simulink model "fw_vehicle_ctrl"  (R2026b)
settings: Solver=VariableStepAuto
undefined symbols (not defined in the file or in its folder): DiscIntNeverNeededParam, ImplementType, P, ShaddadMode, Ts
libraries: simulink x22, sl_discontinuities x6, slpidlib x1
settings Model: Creator=aomar  LastModifiedBy=aomar

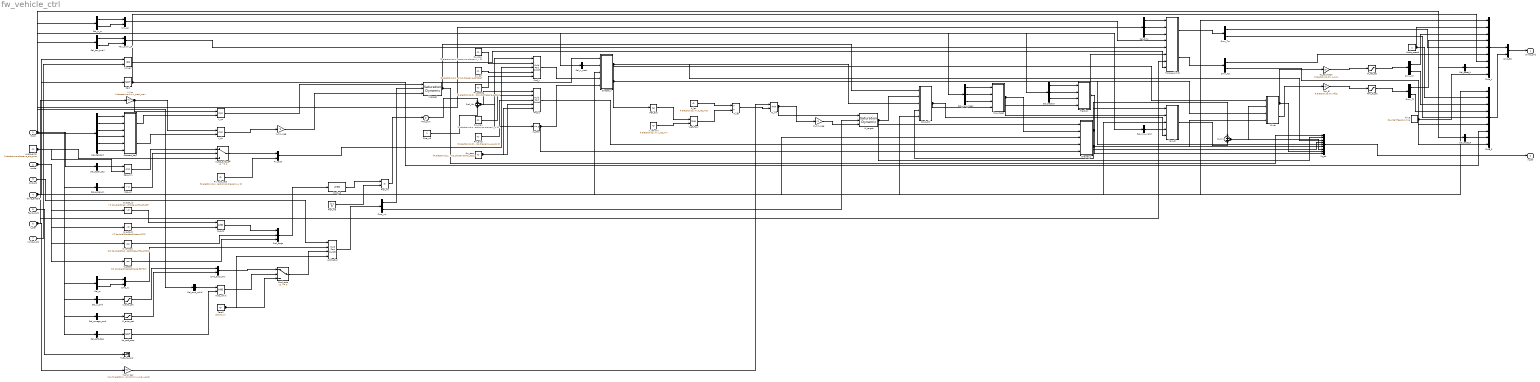
== system fw_vehicle_ctrl ==
  fw10 : Inport  SampleTime=Ts.ctrl
  mode : Inport  Port=2  OutDataTypeStr=uint8  SampleTime=Ts.ctrl
  cmd_src : Inport  Port=3  OutDataTypeStr=uint8  SampleTime=Ts.ctrl
  drive_enable : Inport  Port=4  OutDataTypeStr=boolean  SampleTime=Ts.ctrl
  fault_word : Inport  Port=5  OutDataTypeStr=uint32  SampleTime=Ts.ctrl
  k_der : Inport  Port=6  OutDataTypeStr=single  SampleTime=Ts.ctrl
  limits_hold : Inport  Port=7  OutDataTypeStr=boolean  SampleTime=Ts.ctrl
  A_acc_auto : Constant  Value=P.electronics.shaper.a_acc_auto  OutDataTypeStr=single  SampleTime=Ts.ctrl
  A_acc_auto_eff : Switch  Criteria=u2 ~= 0  SaturateOnIntegerOverflow=off  InputSameDT=off
  A_lat : Constant  Value=P.electronics.lim.a_lat_max  OutDataTypeStr=single  SampleTime=Ts.ctrl
  Alive : simulink/Sources/Counter Free-Running  NumBits=8  tsamp=Ts.ctrl
  Arbitration : MultiPortSwitch  DataPortOrder=Specify indices  DataPortIndices={1,2}  DataPortForDefault=Additional data port  DiagnosticForDefault=None  SaturateOnIntegerOverflow=off  InputSameDT=off
  Auto_valid : Logic  AllPortsSameDT=off  OutDataTypeStr=boolean
  Cap_min : MinMax  Inputs=2
  Cap_on : simulink/Logic and Bit Operations/Compare To Zero  relop=>  OutDataTypeStr=boolean
  Cmd_BC : BusCreator  Inputs=2  OutDataTypeStr=Bus: Bus_DriveCmd  NonVirtualBus=on
      settings: InheritFromInputs=off
  Cmd_auto : Switch  Criteria=u2 ~= 0  SaturateOnIntegerOverflow=off  InputSameDT=off
  Cmd_auto_raw : Concatenate
  Cmd_rc : Concatenate
  Cmd_still : Subsystem
  Cmd_vw : Demux  Outputs=2
  Descent_cap : Subsystem
  Dmx_Tf : Demux  Outputs=2
  Dmx_Tg : Demux  Outputs=2
  Dmx_Tm : Demux  Outputs=2
  Dmx_Wr : Demux  Outputs=2
  Is_auto : Logic  AllPortsSameDT=off  OutDataTypeStr=boolean
  Is_auto_hi : simulink/Logic and Bit Operations/Compare To Constant  relop=<=  const=double(ShaddadMode.AUTO)  OutDataTypeStr=boolean
  Is_auto_lo : simulink/Logic and Bit Operations/Compare To Constant  relop=>=  const=double(ShaddadMode.AUTO_START)  OutDataTypeStr=boolean
  Is_ctrlstop : simulink/Logic and Bit Operations/Compare To Constant  relop===  const=double(ShaddadMode.CTRL_STOP)  OutDataTypeStr=boolean
  Is_estop : simulink/Logic and Bit Operations/Compare To Constant  relop===  const=double(ShaddadMode.ESTOP)  OutDataTypeStr=boolean
  Is_stop : simulink/Logic and Bit Operations/Compare To Constant  relop=>=  const=3  OutDataTypeStr=boolean
  Lim_en : Logic  Operator=OR  AllPortsSameDT=off  OutDataTypeStr=boolean
  Mixer : Subsystem
  Mode_speed : Constant  OutDataTypeStr=uint8  SampleTime=Ts.ctrl
  No_soft_stop : Logic  Operator=NOT  Inputs=1  AllPortsSameDT=off  OutDataTypeStr=boolean
  One_u8 : Constant  OutDataTypeStr=uint8  SampleTime=Ts.ctrl
  Park : Logic  Operator=NOT  Inputs=1  AllPortsSameDT=off  OutDataTypeStr=boolean
  Prof_flags : Concatenate  NumInputs=3
  Prof_idx : Sum  OutDataTypeStr=uint8
  Prof_sum : Sum  Inputs=+  OutDataTypeStr=uint8
  Prof_u8 : DataTypeConversion  OutDataTypeStr=uint8  RndMeth=Round
  Prof_v : MultiPortSwitch  Inputs=4  DiagnosticForDefault=None  SaturateOnIntegerOverflow=off  InputSameDT=off
  Prof_w : MultiPortSwitch  Inputs=4  DiagnosticForDefault=None  SaturateOnIntegerOverflow=off  InputSameDT=off
  Prof_w8 : Constant  Value=[1 2 3]  OutDataTypeStr=uint8  SampleTime=Ts.ctrl
  Prof_wt : Product  Inputs=**  OutDataTypeStr=uint8
  Pv_auto : Concatenate
  Pv_auto_rest : Constant  Value=[P.electronics.shaper.a_dec_auto P.electronics.shaper.j_max P.electronics.shaper.K_v 0]  OutDataTypeStr=single  SampleTime=Ts.ctrl
  Pv_ctrl : Constant  Value=[P.electronics.shaper.a_ctrlstop P.electronics.shaper.a_ctrlstop P.electronics.shaper.j_stop P.electronics.shaper.K_v P.electronics.shaper.a_ctrlstop]  OutDataTypeStr=single  SampleTime=Ts.ctrl
  Pv_estop : Constant  Value=[P.electronics.shaper.a_estop P.electronics.shaper.a_estop P.electronics.shaper.j_stop P.electronics.shaper.K_v P.electronics.shaper.a_estop]  OutDataTypeStr=single  SampleTime=Ts.ctrl
  Pv_man : Constant  Value=[P.electronics.shaper.a_acc_man P.electronics.shaper.a_dec_man P.electronics.shaper.j_max P.electronics.shaper.K_v 0]  OutDataTypeStr=single  SampleTime=Ts.ctrl
  Pw_auto : Constant  Value=[P.electronics.shaper.alpha_auto P.electronics.shaper.alpha_auto P.electronics.shaper.jw_auto P.electronics.shaper.K_w_auto 0]  OutDataTypeStr=single  SampleTime=Ts.ctrl
  Pw_man : Constant  Value=[P.electronics.shaper.alpha_max P.electronics.shaper.alpha_max P.electronics.shaper.jw_max P.electronics.shaper.K_w 0]  OutDataTypeStr=single  SampleTime=Ts.ctrl
  Pw_stop : Constant  Value=[P.electronics.shaper.alpha_stop P.electronics.shaper.alpha_stop P.electronics.shaper.jw_stop P.electronics.shaper.K_w P.electronics.shaper.alpha_stop]  OutDataTypeStr=single  SampleTime=Ts.ctrl
  Sel_accel_cap : BusSelector  OutputSignals=gnc_cmd.accel_limit
  Sel_accel_on : BusSelector  OutputSignals=gnc_cmd.accel_limit
  Sel_bms : BusSelector  OutputSignals=bms.V_pack,bms.DCL,bms.CCL
  Sel_cmd_valid : BusSelector  OutputSignals=gnc_cmd.cmd_valid
  Sel_descent : BusSelector  OutputSignals=tilt.pitch,tilt.imu_valid,di_word,impl.impl_type,impl.rx_ok,adc.lift_pos
  Sel_imu_valid : BusSelector  OutputSignals=tilt.imu_valid
  Sel_omega_cmd : BusSelector  OutputSignals=gnc_cmd.omega_cmd
  Sel_rc : BusSelector  OutputSignals=rc.v_rc,rc.w_rc
  Sel_reset_L : BusSelector  OutputSignals=reset_req
  Sel_reset_R : BusSelector  OutputSignals=reset_req
  Sel_soft_stop : BusSelector  OutputSignals=gnc_cmd.soft_stop_req
  Sel_tau_avail : BusSelector  OutputSignals=drive_fb.L.tau_avail,drive_fb.R.tau_avail
  Sel_traction : BusSelector  OutputSignals=odom.vTrack_LR,gnc_cmd.v_ground_est,gnc_cmd.v_ground_valid
  Sel_v_cmd : BusSelector  OutputSignals=gnc_cmd.v_cmd
  Sel_v_track : BusSelector  OutputSignals=v_track
  Sel_w_m : BusSelector  OutputSignals=drive_fb.L.w_m,drive_fb.R.w_m
  Sel_yaw_meas : BusSelector  OutputSignals=tilt.yaw_rate_meas,tilt.gyro_bias,odom.vTrack_LR
  Shaper_v : Subsystem
  Shaper_w : Subsystem
  Side_L : BusCreator  Inputs=9  OutDataTypeStr=Bus: Bus_DriveSideCmd  NonVirtualBus=on
      settings: InheritFromInputs=off
  Side_R : BusCreator  Inputs=9  OutDataTypeStr=Bus: Bus_DriveSideCmd  NonVirtualBus=on
      settings: InheritFromInputs=off
  T_fault_word : Terminator
  Tau_avail_LR : Concatenate
  Tau_ff : Gain  Gain=P.electronics.drv.Kff_a
  Tau_ff_sat : Saturate  UpperLimit=P.electronics.drv.T_peak  LowerLimit=-P.electronics.drv.T_peak
  Torque_Limits : Subsystem
  Traction : Subsystem
  V_auto_sat : Saturate  UpperLimit=P.electronics.lim.v_max_auto  LowerLimit=-P.electronics.lim.v_rev_auto
  V_dn : MinMax  Inputs=2
  V_lat_min : Constant  Value=P.electronics.lim.v_lat_min  OutDataTypeStr=single  SampleTime=Ts.ctrl
  V_lim : Gain  Gain=P.electronics.lim.v_track_max
  V_lim_neg : Gain  Gain=-1
  V_target : sl_discontinuities/Saturation Dynamic  OutMin=[]  OutMax=[]  OutDataTypeStr=Inherit: Same as second input  OutDataType=fixdt(1, 16)  OutScaling=2^-10  DoSatur=off
      settings: LibrarySourceBlock=|
      | simulink/Discontinuities/Saturation
      | Dynamic
  V_up : MinMax  Inputs=2
  Vc_tel : Concatenate  NumInputs=9
  Vref_abs : Abs  SaturateOnIntegerOverflow=off
  Vref_floor : MinMax  Function=max  Inputs=2
  W_auto_sat : Saturate  UpperLimit=P.electronics.lim.w_max_auto  LowerLimit=-P.electronics.lim.w_max_auto
  W_lat : Product  Inputs=*/
  W_lim : MinMax  Inputs=2
  W_lim_der : Gain  Gain=max(P.electronics.lim.w_max_man, P.electronics.lim.w_max_auto)
  W_lim_neg : Gain  Gain=-1
  W_mix : Sum
  W_ref_motor : Gain  Gain=P.electronics.drv.k_v2w
  W_ref_sat : Saturate  UpperLimit=P.electronics.drv.w_ref_max  LowerLimit=-P.electronics.drv.w_ref_max
  W_target : sl_discontinuities/Saturation Dynamic  OutMin=[]  OutMax=[]  OutDataTypeStr=Inherit: Same as second input  OutDataType=fixdt(1, 16)  OutScaling=2^-10  DoSatur=off
      settings: LibrarySourceBlock=|
      | simulink/Discontinuities/Saturation
      | Dynamic
  Wm_LR : Concatenate
  Yaw_PI : Subsystem
  Yaw_meas : Subsystem
  Zero2 : Constant  Value=zeros(1,2)  OutDataTypeStr=single  SampleTime=Ts.ctrl
  drive_cmd : Outport  OutDataTypeStr=Bus: Bus_DriveCmd
  vc_tel : Outport  Port=2  OutDataTypeStr=single
  wires:
  fw10/1 -> Sel_soft_stop/1, Sel_omega_cmd/1, Sel_v_cmd/1, Sel_cmd_valid/1, Sel_rc/1, Sel_w_m/1, Sel_bms/1, Sel_tau_avail/1, Sel_v_track/1, Sel_reset_L/1, Sel_accel_on/1, Sel_traction/1, Sel_yaw_meas/1, Sel_accel_cap/1, Sel_reset_R/1, Sel_imu_valid/1, Sel_descent/1  "fw10"
  A_acc_auto/1 -> Cap_min/2, A_acc_auto_eff/3  "A_acc_auto"
  mode/1 -> Is_estop/1, Is_ctrlstop/1, Is_auto_hi/1, Is_auto_lo/1  "mode"
  cmd_src/1 -> Arbitration/1  "cmd_src"
  drive_enable/1 -> Side_L/1, Lim_en/1, Shaper_v/3(en), Park/1, Side_R/1, Cmd_still/5(drive_enable), Yaw_PI/3(enable), Shaper_w/3(en)  "drive_enable"
  fault_word/1 -> T_fault_word/1  "fault_word"
  k_der/1 -> Torque_Limits/7(k_der), W_lim_der/1, V_lim/1  "k_der"
  limits_hold/1 -> Lim_en/2  "limits_hold"
  Sel_w_m/1 -> Wm_LR/1  "<w_m>"
  Sel_w_m/2 -> Wm_LR/2  "<w_m>"
  Sel_tau_avail/1 -> Tau_avail_LR/1  "<tau_avail>"
  Sel_tau_avail/2 -> Tau_avail_LR/2  "<tau_avail>"
  Sel_descent/1 -> Descent_cap/1(pitch)  "<pitch>"
  Sel_descent/2 -> Descent_cap/2(imu_valid)  "<imu_valid>"
  Sel_descent/3 -> Descent_cap/3(di_word)  "<di_word>"
  Sel_descent/4 -> Descent_cap/4(impl_type)  "<impl_type>"
  Sel_descent/5 -> Descent_cap/5(impl_rx_ok)  "<rx_ok>"
  Sel_descent/6 -> Descent_cap/6(lift_pos)  "<lift_pos>"
  Sel_accel_cap/1 -> Cap_min/1  "<accel_limit>"
  Sel_accel_on/1 -> Cap_on/1  "<accel_limit>"
  Sel_rc/1 -> Cmd_rc/1  "<v_rc>"
  Sel_rc/2 -> Cmd_rc/2  "<w_rc>"
  Sel_v_cmd/1 -> V_auto_sat/1  "<v_cmd>"
  Sel_omega_cmd/1 -> W_auto_sat/1  "<omega_cmd>"
  Sel_soft_stop/1 -> No_soft_stop/1  "<soft_stop_req>"
  Wm_LR/1 -> Torque_Limits/4(w_m)  "w_m"
  Tau_avail_LR/1 -> Torque_Limits/5(tau_avail)  "tau_avail"
  Cmd_rc/1 -> Arbitration/2  "Cmd_rc"
  Lim_en/1 -> Torque_Limits/8(enable)  "limits_on"
  Park/1 -> Side_R/7, Side_L/7  "park_req"
  Cap_min/1 -> A_acc_auto_eff/1  "Cap_min"
  Cap_on/1 -> A_acc_auto_eff/2  "Cap_on"
  Is_auto_lo/1 -> Is_auto/1  "Is_auto_lo"
  Is_auto_hi/1 -> Is_auto/2  "Is_auto_hi"
  Is_ctrlstop/1 -> Prof_flags/2  "Is_ctrlstop"
  Is_estop/1 -> Prof_flags/3  "Is_estop"
  V_auto_sat/1 -> Cmd_auto_raw/1  "V_auto_sat"
  W_auto_sat/1 -> Cmd_auto_raw/2  "W_auto_sat"
  No_soft_stop/1 -> Auto_valid/2  "No_soft_stop"
  W_lim_der/1 -> W_lim/1  "W_lim_der"
  V_lim/1 -> V_dn/1, V_up/1  "v_lim"
  Descent_cap/1(ref_fwd) -> V_up/2  "ref_fwd"
  Descent_cap/2(ref_rev) -> V_dn/2  "ref_rev"
  Sel_cmd_valid/1 -> Auto_valid/1  "<cmd_valid>"
  Cmd_auto_raw/1 -> Cmd_auto/1  "Cmd_auto_raw"
  V_up/1 -> V_target/1  "v_up"
  V_dn/1 -> V_lim_neg/1  "v_dn"
  Pv_auto_rest/1 -> Pv_auto/2  "Pv_auto_rest"
  Is_auto/1 -> Prof_flags/1  "Is_auto"
  Auto_valid/1 -> Cmd_auto/2  "Auto_valid"
  Zero2/1 -> Arbitration/4, Cmd_auto/3  "Zero2"
  A_acc_auto_eff/1 -> Pv_auto/1  "a_acc_auto"
  Pv_auto/1 -> Prof_v/3  "Pv_auto"
  Prof_flags/1 -> Prof_u8/1  "Prof_flags"
  V_lim_neg/1 -> V_target/3  "V_lim_neg"
  Cmd_auto/1 -> Arbitration/3  "Cmd_auto"
  Prof_w8/1 -> Prof_wt/2  "Prof_w8"
  Arbitration/1 -> Cmd_vw/1  "cmd_sel"
  Prof_u8/1 -> Prof_wt/1  "Prof_u8"
  Cmd_vw/1 -> V_target/2  "v_sel"
  Cmd_vw/2 -> W_target/2  "w_sel"
  Prof_wt/1 -> Prof_sum/1  "Prof_wt"
  Prof_sum/1 -> Prof_idx/1  "Prof_sum"
  One_u8/1 -> Prof_idx/2  "One_u8"
  V_target/1 -> Vc_tel/1, Shaper_v/1(x_t), Cmd_still/1(v_target)  "v_target"
  Prof_idx/1 -> Prof_v/1, Is_stop/1, Prof_w/1  "profile"
  Pv_man/1 -> Prof_v/2  "Pv_man"
  Pv_ctrl/1 -> Prof_v/4  "Pv_ctrl"
  Pv_estop/1 -> Prof_v/5  "Pv_estop"
  Pw_man/1 -> Prof_w/2  "Pw_man"
  Pw_auto/1 -> Prof_w/3  "Pw_auto"
  Pw_stop/1 -> Prof_w/4, Prof_w/5  "Pw_stop"
  Is_stop/1 -> Shaper_v/5(is_stop), Shaper_w/5(is_stop)  "is_stop"
  Prof_v/1 -> Shaper_v/4(prof)  "prof_v"
  Prof_w/1 -> Shaper_w/4(prof)  "prof_w"
  Sel_v_track/1 -> Shaper_v/2(x_meas)  "<v_track>"
  Shaper_v/1(x_ref) -> Vc_tel/3, Vref_abs/1, Cmd_still/3(v_ref), Mixer/1(v_ref)  "v_ref"
  Shaper_v/2(a_ref) -> Vc_tel/5, Mixer/3(a_ref)  "a_ref"
  Vref_abs/1 -> Vref_floor/1  "Vref_abs"
  V_lat_min/1 -> Vref_floor/2  "V_lat_min"
  A_lat/1 -> W_lat/1  "A_lat"
  Vref_floor/1 -> W_lat/2  "Vref_floor"
  W_lat/1 -> W_lim/2  "W_lat"
  W_lim/1 -> W_lim_neg/1, W_target/1  "w_lim"
  W_lim_neg/1 -> W_target/3  "W_lim_neg"
  W_target/1 -> Cmd_still/2(w_target), Vc_tel/2, Shaper_w/1(x_t)  "w_target"
  Cmd_still/1(cmd_still) -> Yaw_PI/5(cmd_still), Yaw_meas/4(cmd_still)  "cmd_still"
  Sel_yaw_meas/1 -> Yaw_meas/1(yaw_rate_meas)  "<yaw_rate_meas>"
  Sel_yaw_meas/2 -> Yaw_meas/2(gyro_bias)  "<gyro_bias>"
  Sel_yaw_meas/3 -> Yaw_meas/3(v_track_LR)  "<vTrack_LR>"
  Yaw_meas/1(yaw_rate) -> Shaper_w/2(x_meas), Yaw_PI/2(yaw_meas), Traction/4(yaw_rate)  "yaw_rate_meas"
  Sel_traction/1 -> Traction/1(v_track_LR)  "<vTrack_LR>"
  Sel_traction/2 -> Traction/2(v_ground)  "<v_ground_est>"
  Sel_traction/3 -> Traction/3(v_ground_valid)  "<v_ground_valid>"
  Traction/1(k_tr) -> Vc_tel/9, Torque_Limits/6(k_tr)  "k_tr"
  Shaper_w/1(x_ref) -> Yaw_PI/1(w_ref), Cmd_still/4(w_ref), Vc_tel/4, W_mix/1  "w_ref"
  Shaper_w/2(a_ref) -> Mixer/4(alpha_ref), Vc_tel/6  "alpha_ref"
  Sel_bms/1 -> Torque_Limits/1(V_pack)  "<V_pack>"
  Sel_bms/2 -> Torque_Limits/2(DCL)  "<DCL>"
  Sel_bms/3 -> Torque_Limits/3(CCL)  "<CCL>"
  Sel_imu_valid/1 -> Yaw_PI/4(imu_valid)  "<imu_valid>"
  Torque_Limits/1(tau_lim_mot) -> Dmx_Tm/1  "tau_lim_mot_LR"
  Torque_Limits/2(tau_lim_reg) -> Dmx_Tg/1  "tau_lim_reg_LR"
  Yaw_PI/1(u) -> W_mix/2  "u_yaw"
  Dmx_Tm/1 -> Side_L/5  "tau_lim_mot"
  Dmx_Tm/2 -> Side_R/5  "tau_lim_mot"
  Dmx_Tg/1 -> Side_L/6  "tau_lim_reg"
  Dmx_Tg/2 -> Side_R/6  "tau_lim_reg"
  W_mix/1 -> Mixer/2(w_mix), Vc_tel/7  "w_mix"
  Mixer/1(vtrack_ref) -> Vc_tel/8, W_ref_motor/1  "vtrack_ref"
  Mixer/2(atrack_ref) -> Tau_ff/1  "atrack_ref"
  Vc_tel/1 -> vc_tel/1  "vc_tel"
  W_ref_motor/1 -> W_ref_sat/1  "W_ref_motor"
  Tau_ff/1 -> Tau_ff_sat/1  "Tau_ff"
  W_ref_sat/1 -> Dmx_Wr/1  "w_ref_LR"
  Tau_ff_sat/1 -> Dmx_Tf/1  "tau_ff_LR"
  Dmx_Wr/1 -> Side_L/3  "w_ref"
  Dmx_Wr/2 -> Side_R/3  "w_ref"
  Dmx_Tf/1 -> Side_L/4  "tau_ff"
  Dmx_Tf/2 -> Side_R/4  "tau_ff"
  Mode_speed/1 -> Side_R/2, Side_L/2  "mode"
  Alive/1 -> Side_L/9, Side_R/9  "alive"
  Sel_reset_L/1 -> Side_L/8  "<reset_req>"
  Sel_reset_R/1 -> Side_R/8  "<reset_req>"
  Side_L/1 -> Cmd_BC/1  "L"
  Side_R/1 -> Cmd_BC/2  "R"
  Cmd_BC/1 -> drive_cmd/1  "drive_cmd"

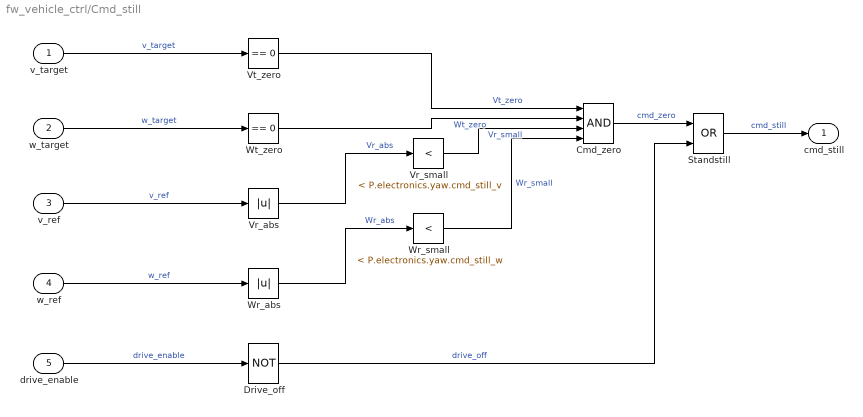
== system fw_vehicle_ctrl/Cmd_still ==
  v_target : Inport
  w_target : Inport  Port=2
  v_ref : Inport  Port=3
  w_ref : Inport  Port=4
  drive_enable : Inport  Port=5
  Cmd_zero : Logic  Inputs=4  AllPortsSameDT=off  OutDataTypeStr=boolean
  Drive_off : Logic  Operator=NOT  Inputs=1  AllPortsSameDT=off  OutDataTypeStr=boolean
  Standstill : Logic  Operator=OR  AllPortsSameDT=off  OutDataTypeStr=boolean
  Vr_abs : Abs  SaturateOnIntegerOverflow=off
  Vr_small : simulink/Logic and Bit Operations/Compare To Constant  relop=<  const=P.electronics.yaw.cmd_still_v  OutDataTypeStr=boolean
  Vt_zero : simulink/Logic and Bit Operations/Compare To Zero  relop===  OutDataTypeStr=boolean
  Wr_abs : Abs  SaturateOnIntegerOverflow=off
  Wr_small : simulink/Logic and Bit Operations/Compare To Constant  relop=<  const=P.electronics.yaw.cmd_still_w  OutDataTypeStr=boolean
  Wt_zero : simulink/Logic and Bit Operations/Compare To Zero  relop===  OutDataTypeStr=boolean
  cmd_still : Outport
  wires:
  v_target/1 -> Vt_zero/1  "v_target"
  w_target/1 -> Wt_zero/1  "w_target"
  v_ref/1 -> Vr_abs/1  "v_ref"
  w_ref/1 -> Wr_abs/1  "w_ref"
  drive_enable/1 -> Drive_off/1  "drive_enable"
  Vt_zero/1 -> Cmd_zero/1  "Vt_zero"
  Wt_zero/1 -> Cmd_zero/2  "Wt_zero"
  Vr_abs/1 -> Vr_small/1  "Vr_abs"
  Wr_abs/1 -> Wr_small/1  "Wr_abs"
  Drive_off/1 -> Standstill/2  "drive_off"
  Vr_small/1 -> Cmd_zero/3  "Vr_small"
  Wr_small/1 -> Cmd_zero/4  "Wr_small"
  Cmd_zero/1 -> Standstill/1  "cmd_zero"
  Standstill/1 -> cmd_still/1  "cmd_still"

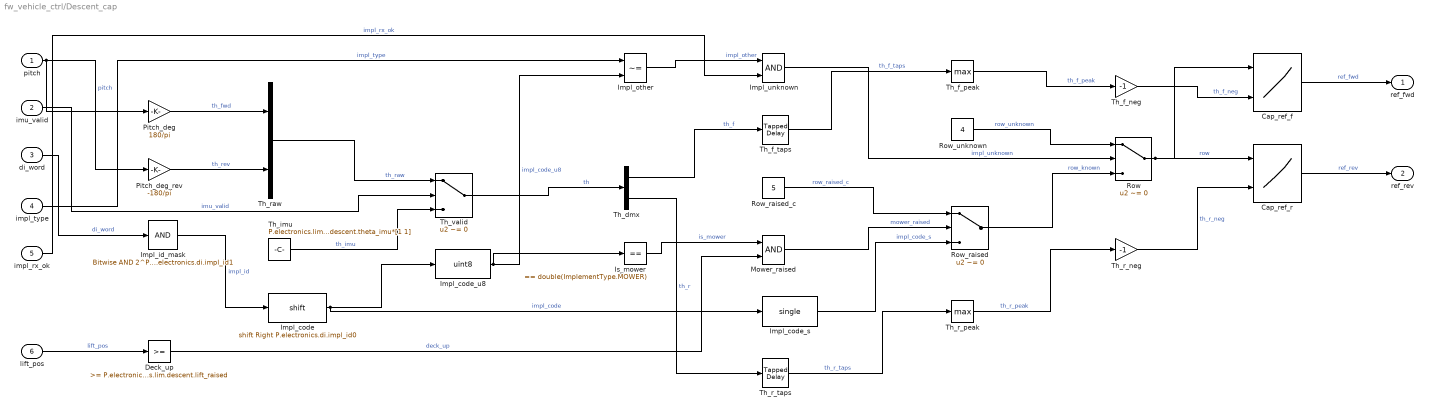
== system fw_vehicle_ctrl/Descent_cap ==
  pitch : Inport
  imu_valid : Inport  Port=2
  di_word : Inport  Port=3
  impl_type : Inport  Port=4
  impl_rx_ok : Inport  Port=5
  lift_pos : Inport  Port=6
  Cap_ref_f : Lookup_n-D  BreakpointsForDimension1=0:5  BreakpointsForDimension2=-fliplr(P.electronics.lim.descent.theta_bp)  BreakpointsForDimension1DataTypeStr=single  BreakpointsForDimension2DataTypeStr=single  Table=P.electronics.lim.descent.ref_fwd(:, end:-1:1)  TableDataTypeStr=single  InterpMethod=Flat  ExtrapMethod=Clip  InternalRulePriority=Speed  OutDataTypeStr=single  RndMeth=Simplest
      settings: InputPortMap=u0,u1
  Cap_ref_r : Lookup_n-D  BreakpointsForDimension1=0:5  BreakpointsForDimension2=-fliplr(P.electronics.lim.descent.theta_bp)  BreakpointsForDimension1DataTypeStr=single  BreakpointsForDimension2DataTypeStr=single  Table=P.electronics.lim.descent.ref_rev(:, end:-1:1)  TableDataTypeStr=single  InterpMethod=Flat  ExtrapMethod=Clip  InternalRulePriority=Speed  OutDataTypeStr=single  RndMeth=Simplest
      settings: InputPortMap=u0,u1
  Deck_up : simulink/Logic and Bit Operations/Compare To Constant  relop=>=  const=P.electronics.lim.descent.lift_raised  OutDataTypeStr=boolean
  Impl_code : ArithShift  BitShiftNumber=P.electronics.di.impl_id0  BitShiftDirection=Right
  Impl_code_s : DataTypeConversion  OutDataTypeStr=single  RndMeth=Round
  Impl_code_u8 : DataTypeConversion  OutDataTypeStr=uint8  RndMeth=Round
  Impl_id_mask : simulink/Logic and Bit Operations/Bitwise Operator  logicop=AND  UseBitMask=on  BitMask=2^P.electronics.di.impl_id0 + 2^P.electronics.di.impl_id1  BitMaskRealWorld=Stored Integer
  Impl_other : RelationalOperator  Operator=~=  OutDataTypeStr=boolean  RndMeth=Simplest  InputSameDT=off
  Impl_unknown : Logic  AllPortsSameDT=off  OutDataTypeStr=boolean
  Is_mower : simulink/Logic and Bit Operations/Compare To Constant  relop===  const=double(ImplementType.MOWER)  OutDataTypeStr=boolean
  Mower_raised : Logic  AllPortsSameDT=off  OutDataTypeStr=boolean
  Pitch_deg : Gain  Gain=180/pi
  Pitch_deg_rev : Gain  Gain=-180/pi
  Row : Switch  Criteria=u2 ~= 0  SaturateOnIntegerOverflow=off  InputSameDT=off
  Row_raised : Switch  Criteria=u2 ~= 0  SaturateOnIntegerOverflow=off  InputSameDT=off
  Row_raised_c : Constant  Value=5  OutDataTypeStr=single  SampleTime=Ts.ctrl
  Row_unknown : Constant  Value=4  OutDataTypeStr=single  SampleTime=Ts.ctrl
  Th_dmx : Demux  Outputs=2
  Th_f_neg : Gain  Gain=-1
  Th_f_peak : MinMax  Function=max
  Th_f_taps : simulink/Discrete/Tapped Delay  vinit=P.electronics.lim.descent.theta_imu  samptime=-1  NumDelays=round(P.electronics.lim.descent.t_hold/Ts.ctrl) - 1  DelayOrder=Oldest  includeCurrent=on
  Th_imu : Constant  Value=P.electronics.lim.descent.theta_imu*[1 1]  OutDataTypeStr=single  SampleTime=Ts.ctrl
  Th_r_neg : Gain  Gain=-1
  Th_r_peak : MinMax  Function=max
  Th_r_taps : simulink/Discrete/Tapped Delay  vinit=P.electronics.lim.descent.theta_imu  samptime=-1  NumDelays=round(P.electronics.lim.descent.t_hold/Ts.ctrl) - 1  DelayOrder=Oldest  includeCurrent=on
  Th_raw : Concatenate
  Th_valid : Switch  Criteria=u2 ~= 0  SaturateOnIntegerOverflow=off  InputSameDT=off
  ref_fwd : Outport
  ref_rev : Outport  Port=2
  wires:
  pitch/1 -> Pitch_deg_rev/1, Pitch_deg/1  "pitch"
  imu_valid/1 -> Th_valid/2  "imu_valid"
  di_word/1 -> Impl_id_mask/1  "di_word"
  impl_type/1 -> Impl_other/1  "impl_type"
  impl_rx_ok/1 -> Impl_unknown/2  "impl_rx_ok"
  lift_pos/1 -> Deck_up/1  "lift_pos"
  Pitch_deg/1 -> Th_raw/1  "th_fwd"
  Pitch_deg_rev/1 -> Th_raw/2  "th_rev"
  Deck_up/1 -> Mower_raised/2  "deck_up"
  Impl_id_mask/1 -> Impl_code/1  "impl_id"
  Th_raw/1 -> Th_valid/1  "th_raw"
  Th_imu/1 -> Th_valid/3  "th_imu"
  Impl_code/1 -> Impl_code_u8/1, Impl_code_s/1  "impl_code"
  Th_valid/1 -> Th_dmx/1  "th"
  Impl_code_u8/1 -> Impl_other/2, Is_mower/1  "impl_code_u8"
  Th_dmx/1 -> Th_f_taps/1  "th_f"
  Th_dmx/2 -> Th_r_taps/1  "th_r"
  Impl_other/1 -> Impl_unknown/1  "impl_other"
  Is_mower/1 -> Mower_raised/1  "is_mower"
  Impl_unknown/1 -> Row/2  "impl_unknown"
  Row_raised_c/1 -> Row_raised/1  "row_raised_c"
  Mower_raised/1 -> Row_raised/2  "mower_raised"
  Th_f_taps/1 -> Th_f_peak/1  "th_f_taps"
  Th_r_taps/1 -> Th_r_peak/1  "th_r_taps"
  Impl_code_s/1 -> Row_raised/3  "impl_code_s"
  Th_f_peak/1 -> Th_f_neg/1  "th_f_peak"
  Row_unknown/1 -> Row/1  "row_unknown"
  Th_r_peak/1 -> Th_r_neg/1  "th_r_peak"
  Row_raised/1 -> Row/3  "row_known"
  Th_f_neg/1 -> Cap_ref_f/2  "th_f_neg"
  Th_r_neg/1 -> Cap_ref_r/2  "th_r_neg"
  Row/1 -> Cap_ref_f/1, Cap_ref_r/1  "row"
  Cap_ref_f/1 -> ref_fwd/1  "ref_fwd"
  Cap_ref_r/1 -> ref_rev/1  "ref_rev"

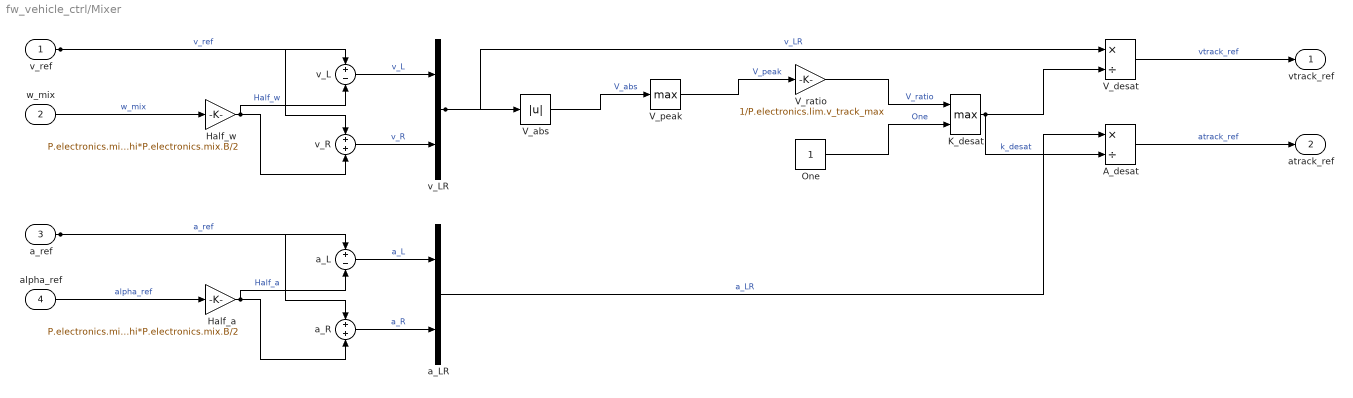
== system fw_vehicle_ctrl/Mixer ==
  v_ref : Inport
  w_mix : Inport  Port=2
  a_ref : Inport  Port=3
  alpha_ref : Inport  Port=4
  A_desat : Product  Inputs=*/
  Half_a : Gain  Gain=P.electronics.mix.chi*P.electronics.mix.B/2
  Half_w : Gain  Gain=P.electronics.mix.chi*P.electronics.mix.B/2
  K_desat : MinMax  Function=max  Inputs=2
  One : Constant  OutDataTypeStr=single  SampleTime=Ts.ctrl
  V_abs : Abs  SaturateOnIntegerOverflow=off
  V_desat : Product  Inputs=*/
  V_peak : MinMax  Function=max
  V_ratio : Gain  Gain=1/P.electronics.lim.v_track_max
  a_L : Sum  Inputs=+-
  a_LR : Concatenate
  a_R : Sum
  v_L : Sum  Inputs=+-
  v_LR : Concatenate
  v_R : Sum
  vtrack_ref : Outport
  atrack_ref : Outport  Port=2
  wires:
  v_ref/1 -> v_R/1, v_L/1  "v_ref"
  w_mix/1 -> Half_w/1  "w_mix"
  a_ref/1 -> a_R/1, a_L/1  "a_ref"
  alpha_ref/1 -> Half_a/1  "alpha_ref"
  Half_w/1 -> v_R/2, v_L/2  "Half_w"
  Half_a/1 -> a_R/2, a_L/2  "Half_a"
  v_L/1 -> v_LR/1  "v_L"
  v_R/1 -> v_LR/2  "v_R"
  a_L/1 -> a_LR/1  "a_L"
  a_R/1 -> a_LR/2  "a_R"
  v_LR/1 -> V_desat/1, V_abs/1  "v_LR"
  a_LR/1 -> A_desat/1  "a_LR"
  V_abs/1 -> V_peak/1  "V_abs"
  V_peak/1 -> V_ratio/1  "V_peak"
  V_ratio/1 -> K_desat/1  "V_ratio"
  One/1 -> K_desat/2  "One"
  K_desat/1 -> V_desat/2, A_desat/2  "k_desat"
  V_desat/1 -> vtrack_ref/1  "vtrack_ref"
  A_desat/1 -> atrack_ref/1  "atrack_ref"

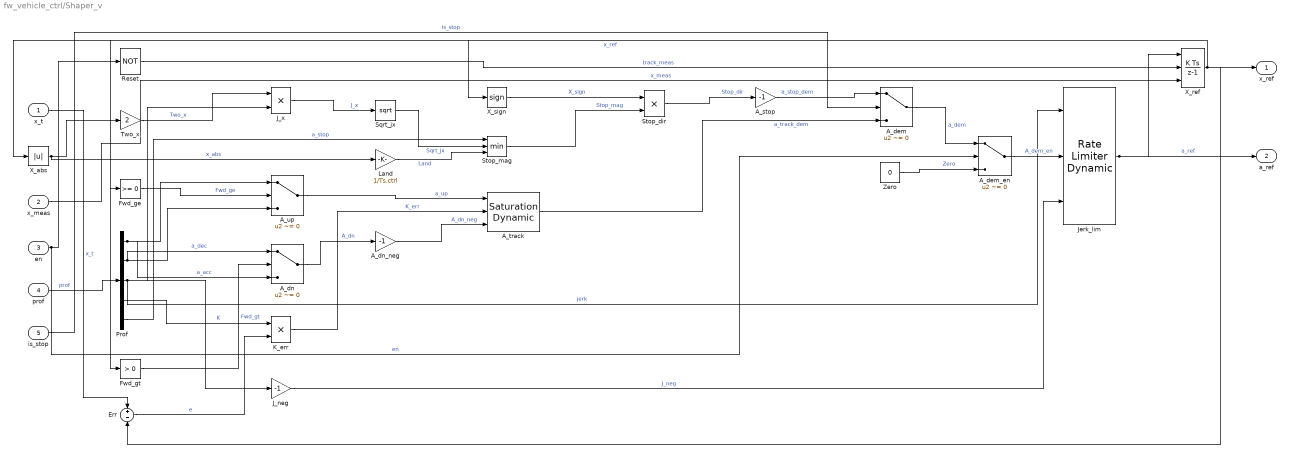
== system fw_vehicle_ctrl/Shaper_v ==
  x_t : Inport
  x_meas : Inport  Port=2
  en : Inport  Port=3
  prof : Inport  Port=4
  is_stop : Inport  Port=5
  A_dem : Switch  Criteria=u2 ~= 0  SaturateOnIntegerOverflow=off  InputSameDT=off
  A_dem_en : Switch  Criteria=u2 ~= 0  SaturateOnIntegerOverflow=off  InputSameDT=off
  A_dn : Switch  Criteria=u2 ~= 0  SaturateOnIntegerOverflow=off  InputSameDT=off
  A_dn_neg : Gain  Gain=-1
  A_stop : Gain  Gain=-1
  A_track : sl_discontinuities/Saturation Dynamic  OutMin=[]  OutMax=[]  OutDataTypeStr=Inherit: Same as second input  OutDataType=fixdt(1, 16)  OutScaling=2^-10  DoSatur=off
      settings: LibrarySourceBlock=|
      | simulink/Discontinuities/Saturation
      | Dynamic
  A_up : Switch  Criteria=u2 ~= 0  SaturateOnIntegerOverflow=off  InputSameDT=off
  Err : Sum  Inputs=+-
  Fwd_ge : simulink/Logic and Bit Operations/Compare To Zero  relop=>=  OutDataTypeStr=boolean
  Fwd_gt : simulink/Logic and Bit Operations/Compare To Zero  relop=>  OutDataTypeStr=boolean
  J_neg : Gain  Gain=-1
  J_x : Product  Inputs=**
  Jerk_lim : sl_discontinuities/Rate Limiter Dynamic
      settings: LibrarySourceBlock=|
      | simulink/Discontinuities/Rate Limiter
      | Dynamic
  K_err : Product  Inputs=**
  Land : Gain  Gain=1/Ts.ctrl
  Prof : Demux  Outputs=5
  Reset : Logic  Operator=NOT  Inputs=1  AllPortsSameDT=off  OutDataTypeStr=boolean
  Sqrt_jx : Sqrt
  Stop_dir : Product  Inputs=**
  Stop_mag : MinMax  Inputs=3
  Two_x : Gain  Gain=2
  X_abs : Abs  SaturateOnIntegerOverflow=off
  X_ref : DiscreteIntegrator  ExternalReset=level  InitialConditionSource=external  SampleTime=-1  ICPrevOutput=DiscIntNeverNeededParam  ICPrevScaledInput=DiscIntNeverNeededParam
  X_sign : Signum
  Zero : Constant  Value=0  OutDataTypeStr=single  SampleTime=Ts.ctrl
  x_ref : Outport
  a_ref : Outport  Port=2
  wires:
  x_t/1 -> Err/1  "x_t"
  X_abs/1 -> Two_x/1, Land/1  "x_abs"
  x_meas/1 -> X_ref/3  "x_meas"
  en/1 -> Reset/1, A_dem_en/2  "en"
  prof/1 -> Prof/1  "prof"
  is_stop/1 -> A_dem/2  "is_stop"
  Prof/3 -> J_x/2, Jerk_lim/1, J_neg/1  "jerk"
  Prof/4 -> K_err/1  "K"
  Prof/5 -> Stop_mag/1  "a_stop"
  Err/1 -> K_err/2  "e"
  Reset/1 -> X_ref/2  "track_meas"
  Two_x/1 -> J_x/1  "Two_x"
  Fwd_ge/1 -> A_up/2  "Fwd_ge"
  Fwd_gt/1 -> A_dn/2  "Fwd_gt"
  J_x/1 -> Sqrt_jx/1  "J_x"
  K_err/1 -> A_track/2  "K_err"
  J_neg/1 -> Jerk_lim/3  "J_neg"
  A_up/1 -> A_track/1  "a_up"
  A_dn/1 -> A_dn_neg/1  "A_dn"
  Sqrt_jx/1 -> Stop_mag/2  "Sqrt_jx"
  Land/1 -> Stop_mag/3  "Land"
  A_dn_neg/1 -> A_track/3  "A_dn_neg"
  X_sign/1 -> Stop_dir/1  "X_sign"
  Stop_mag/1 -> Stop_dir/2  "Stop_mag"
  A_track/1 -> A_dem/3  "a_track_dem"
  Stop_dir/1 -> A_stop/1  "Stop_dir"
  A_stop/1 -> A_dem/1  "a_stop_dem"
  Zero/1 -> A_dem_en/3  "Zero"
  A_dem/1 -> A_dem_en/1  "a_dem"
  A_dem_en/1 -> Jerk_lim/2  "A_dem_en"
  Jerk_lim/1 -> X_ref/1, a_ref/1  "a_ref"
  X_ref/1 -> Err/2, Fwd_gt/1, Fwd_ge/1, X_abs/1, X_sign/1, x_ref/1  "x_ref"
  Prof/1 -> A_up/1, A_dn/3  "a_acc"
  Prof/2 -> A_up/3, A_dn/1  "a_dec"

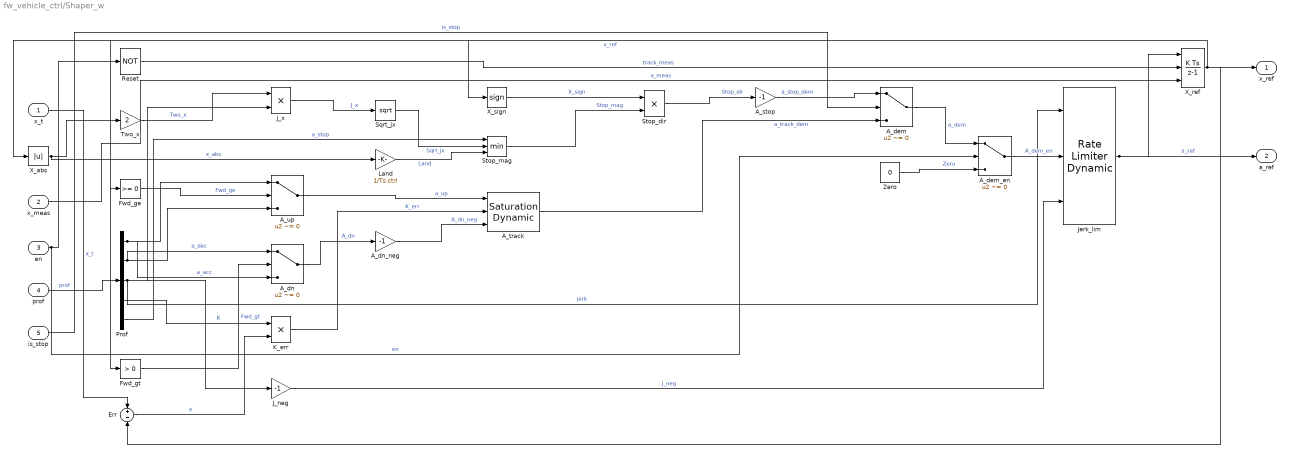
== system fw_vehicle_ctrl/Shaper_w ==
  x_t : Inport
  x_meas : Inport  Port=2
  en : Inport  Port=3
  prof : Inport  Port=4
  is_stop : Inport  Port=5
  A_dem : Switch  Criteria=u2 ~= 0  SaturateOnIntegerOverflow=off  InputSameDT=off
  A_dem_en : Switch  Criteria=u2 ~= 0  SaturateOnIntegerOverflow=off  InputSameDT=off
  A_dn : Switch  Criteria=u2 ~= 0  SaturateOnIntegerOverflow=off  InputSameDT=off
  A_dn_neg : Gain  Gain=-1
  A_stop : Gain  Gain=-1
  A_track : sl_discontinuities/Saturation Dynamic  OutMin=[]  OutMax=[]  OutDataTypeStr=Inherit: Same as second input  OutDataType=fixdt(1, 16)  OutScaling=2^-10  DoSatur=off
      settings: LibrarySourceBlock=|
      | simulink/Discontinuities/Saturation
      | Dynamic
  A_up : Switch  Criteria=u2 ~= 0  SaturateOnIntegerOverflow=off  InputSameDT=off
  Err : Sum  Inputs=+-
  Fwd_ge : simulink/Logic and Bit Operations/Compare To Zero  relop=>=  OutDataTypeStr=boolean
  Fwd_gt : simulink/Logic and Bit Operations/Compare To Zero  relop=>  OutDataTypeStr=boolean
  J_neg : Gain  Gain=-1
  J_x : Product  Inputs=**
  Jerk_lim : sl_discontinuities/Rate Limiter Dynamic
      settings: LibrarySourceBlock=|
      | simulink/Discontinuities/Rate Limiter
      | Dynamic
  K_err : Product  Inputs=**
  Land : Gain  Gain=1/Ts.ctrl
  Prof : Demux  Outputs=5
  Reset : Logic  Operator=NOT  Inputs=1  AllPortsSameDT=off  OutDataTypeStr=boolean
  Sqrt_jx : Sqrt
  Stop_dir : Product  Inputs=**
  Stop_mag : MinMax  Inputs=3
  Two_x : Gain  Gain=2
  X_abs : Abs  SaturateOnIntegerOverflow=off
  X_ref : DiscreteIntegrator  ExternalReset=level  InitialConditionSource=external  SampleTime=-1  ICPrevOutput=DiscIntNeverNeededParam  ICPrevScaledInput=DiscIntNeverNeededParam
  X_sign : Signum
  Zero : Constant  Value=0  OutDataTypeStr=single  SampleTime=Ts.ctrl
  x_ref : Outport
  a_ref : Outport  Port=2
  wires:
  x_t/1 -> Err/1  "x_t"
  X_abs/1 -> Two_x/1, Land/1  "x_abs"
  x_meas/1 -> X_ref/3  "x_meas"
  en/1 -> Reset/1, A_dem_en/2  "en"
  prof/1 -> Prof/1  "prof"
  is_stop/1 -> A_dem/2  "is_stop"
  Prof/3 -> J_x/2, Jerk_lim/1, J_neg/1  "jerk"
  Prof/4 -> K_err/1  "K"
  Prof/5 -> Stop_mag/1  "a_stop"
  Err/1 -> K_err/2  "e"
  Reset/1 -> X_ref/2  "track_meas"
  Two_x/1 -> J_x/1  "Two_x"
  Fwd_ge/1 -> A_up/2  "Fwd_ge"
  Fwd_gt/1 -> A_dn/2  "Fwd_gt"
  J_x/1 -> Sqrt_jx/1  "J_x"
  K_err/1 -> A_track/2  "K_err"
  J_neg/1 -> Jerk_lim/3  "J_neg"
  A_up/1 -> A_track/1  "a_up"
  A_dn/1 -> A_dn_neg/1  "A_dn"
  Sqrt_jx/1 -> Stop_mag/2  "Sqrt_jx"
  Land/1 -> Stop_mag/3  "Land"
  A_dn_neg/1 -> A_track/3  "A_dn_neg"
  X_sign/1 -> Stop_dir/1  "X_sign"
  Stop_mag/1 -> Stop_dir/2  "Stop_mag"
  A_track/1 -> A_dem/3  "a_track_dem"
  Stop_dir/1 -> A_stop/1  "Stop_dir"
  A_stop/1 -> A_dem/1  "a_stop_dem"
  Zero/1 -> A_dem_en/3  "Zero"
  A_dem/1 -> A_dem_en/1  "a_dem"
  A_dem_en/1 -> Jerk_lim/2  "A_dem_en"
  Jerk_lim/1 -> X_ref/1, a_ref/1  "a_ref"
  X_ref/1 -> Err/2, Fwd_gt/1, Fwd_ge/1, X_abs/1, X_sign/1, x_ref/1  "x_ref"
  Prof/1 -> A_up/1, A_dn/3  "a_acc"
  Prof/2 -> A_up/3, A_dn/1  "a_dec"

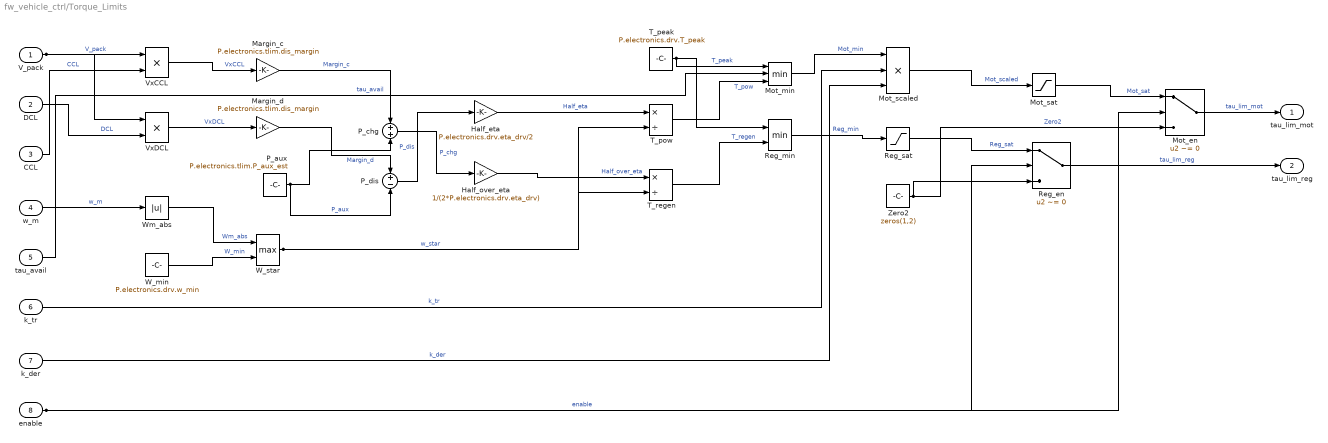
== system fw_vehicle_ctrl/Torque_Limits ==
  V_pack : Inport
  DCL : Inport  Port=2
  CCL : Inport  Port=3
  w_m : Inport  Port=4
  tau_avail : Inport  Port=5
  k_tr : Inport  Port=6
  k_der : Inport  Port=7
  enable : Inport  Port=8
  Half_eta : Gain  Gain=P.electronics.drv.eta_drv/2
  Half_over_eta : Gain  Gain=1/(2*P.electronics.drv.eta_drv)
  Margin_c : Gain  Gain=P.electronics.tlim.dis_margin
  Margin_d : Gain  Gain=P.electronics.tlim.dis_margin
  Mot_en : Switch  Criteria=u2 ~= 0  SaturateOnIntegerOverflow=off  InputSameDT=off
  Mot_min : MinMax  Inputs=3
  Mot_sat : Saturate  UpperLimit=P.electronics.drv.T_peak  LowerLimit=0
  Mot_scaled : Product  Inputs=***
  P_aux : Constant  Value=P.electronics.tlim.P_aux_est  OutDataTypeStr=single  SampleTime=Ts.ctrl
  P_chg : Sum
  P_dis : Sum  Inputs=+-
  Reg_en : Switch  Criteria=u2 ~= 0  SaturateOnIntegerOverflow=off  InputSameDT=off
  Reg_min : MinMax  Inputs=2
  Reg_sat : Saturate  UpperLimit=P.electronics.drv.T_peak  LowerLimit=0
  T_peak : Constant  Value=P.electronics.drv.T_peak  OutDataTypeStr=single  SampleTime=Ts.ctrl
  T_pow : Product  Inputs=*/
  T_regen : Product  Inputs=*/
  VxCCL : Product  Inputs=**
  VxDCL : Product  Inputs=**
  W_min : Constant  Value=P.electronics.drv.w_min  OutDataTypeStr=single  SampleTime=Ts.ctrl
  W_star : MinMax  Function=max  Inputs=2
  Wm_abs : Abs  SaturateOnIntegerOverflow=off
  Zero2 : Constant  Value=zeros(1,2)  OutDataTypeStr=single  SampleTime=Ts.ctrl
  tau_lim_mot : Outport
  tau_lim_reg : Outport  Port=2
  wires:
  V_pack/1 -> VxDCL/1, VxCCL/1  "V_pack"
  DCL/1 -> VxDCL/2  "DCL"
  CCL/1 -> VxCCL/2  "CCL"
  w_m/1 -> Wm_abs/1  "w_m"
  tau_avail/1 -> Mot_min/2  "tau_avail"
  k_tr/1 -> Mot_scaled/2  "k_tr"
  k_der/1 -> Mot_scaled/3  "k_der"
  enable/1 -> Mot_en/2, Reg_en/2  "enable"
  VxCCL/1 -> Margin_c/1  "VxCCL"
  VxDCL/1 -> Margin_d/1  "VxDCL"
  Wm_abs/1 -> W_star/1  "Wm_abs"
  W_min/1 -> W_star/2  "W_min"
  Margin_c/1 -> P_chg/1  "Margin_c"
  Margin_d/1 -> P_dis/1  "Margin_d"
  W_star/1 -> T_pow/2, T_regen/2  "w_star"
  P_aux/1 -> P_chg/2, P_dis/2  "P_aux"
  P_chg/1 -> Half_over_eta/1  "P_chg"
  P_dis/1 -> Half_eta/1  "P_dis"
  Half_eta/1 -> T_pow/1  "Half_eta"
  Half_over_eta/1 -> T_regen/1  "Half_over_eta"
  T_peak/1 -> Reg_min/1, Mot_min/1  "T_peak"
  T_pow/1 -> Mot_min/3  "T_pow"
  T_regen/1 -> Reg_min/2  "T_regen"
  Mot_min/1 -> Mot_scaled/1  "Mot_min"
  Reg_min/1 -> Reg_sat/1  "Reg_min"
  Mot_scaled/1 -> Mot_sat/1  "Mot_scaled"
  Reg_sat/1 -> Reg_en/1  "Reg_sat"
  Zero2/1 -> Mot_en/3, Reg_en/3  "Zero2"
  Mot_sat/1 -> Mot_en/1  "Mot_sat"
  Reg_en/1 -> tau_lim_reg/1  "tau_lim_reg"
  Mot_en/1 -> tau_lim_mot/1  "tau_lim_mot"

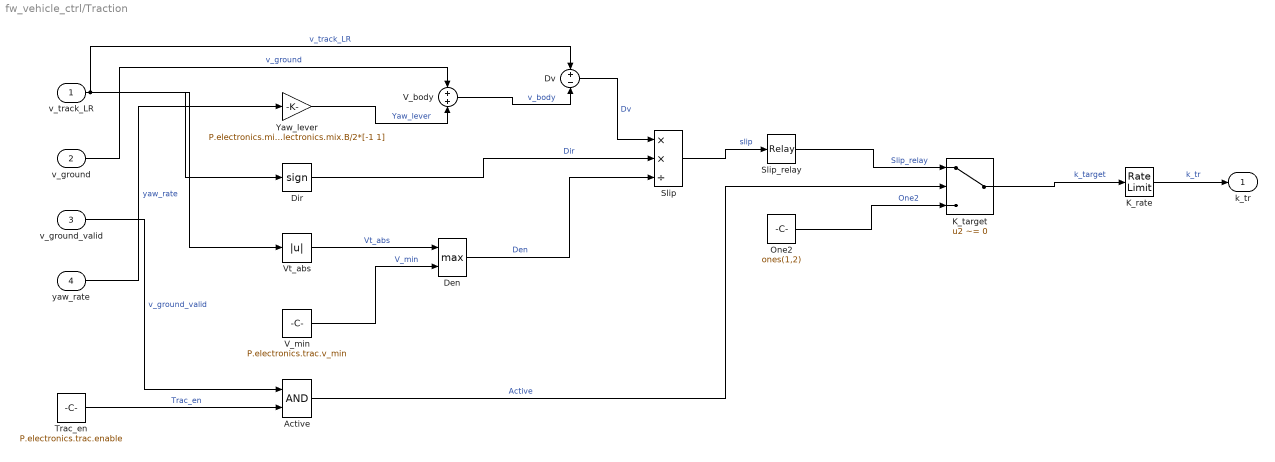
== system fw_vehicle_ctrl/Traction ==
  v_track_LR : Inport
  v_ground : Inport  Port=2
  v_ground_valid : Inport  Port=3
  yaw_rate : Inport  Port=4
  Active : Logic  AllPortsSameDT=off  OutDataTypeStr=boolean
  Den : MinMax  Function=max  Inputs=2
  Dir : Signum
  Dv : Sum  Inputs=+-
  K_rate : RateLimiter  RisingSlewLimit=P.electronics.trac.k_up  FallingSlewLimit=-P.electronics.trac.k_dn  SampleTimeMode=inherited  InitialCondition=1
  K_target : Switch  Criteria=u2 ~= 0  SaturateOnIntegerOverflow=off  InputSameDT=off
  One2 : Constant  Value=ones(1,2)  OutDataTypeStr=single  SampleTime=Ts.ctrl
  Slip : Product  Inputs=**/
  Slip_relay : Relay  OnSwitchValue=P.electronics.trac.s_on  OffSwitchValue=P.electronics.trac.s_off  OnOutputValue=P.electronics.trac.k_min  OffOutputValue=1  OutDataTypeStr=single
  Trac_en : Constant  Value=P.electronics.trac.enable  OutDataTypeStr=boolean  SampleTime=Ts.ctrl
  V_body : Sum
  V_min : Constant  Value=P.electronics.trac.v_min  OutDataTypeStr=single  SampleTime=Ts.ctrl
  Vt_abs : Abs  SaturateOnIntegerOverflow=off
  Yaw_lever : Gain  Gain=P.electronics.mix.chi*P.electronics.mix.B/2*[-1 1]
  k_tr : Outport
  wires:
  v_track_LR/1 -> Vt_abs/1, Dir/1, Dv/1  "v_track_LR"
  v_ground/1 -> V_body/1  "v_ground"
  v_ground_valid/1 -> Active/1  "v_ground_valid"
  yaw_rate/1 -> Yaw_lever/1  "yaw_rate"
  Trac_en/1 -> Active/2  "Trac_en"
  Yaw_lever/1 -> V_body/2  "Yaw_lever"
  Dir/1 -> Slip/2  "Dir"
  Vt_abs/1 -> Den/1  "Vt_abs"
  V_min/1 -> Den/2  "V_min"
  Active/1 -> K_target/2  "Active"
  V_body/1 -> Dv/2  "v_body"
  Den/1 -> Slip/3  "Den"
  Dv/1 -> Slip/1  "Dv"
  Slip/1 -> Slip_relay/1  "slip"
  Slip_relay/1 -> K_target/1  "Slip_relay"
  One2/1 -> K_target/3  "One2"
  K_target/1 -> K_rate/1  "k_target"
  K_rate/1 -> k_tr/1  "k_tr"

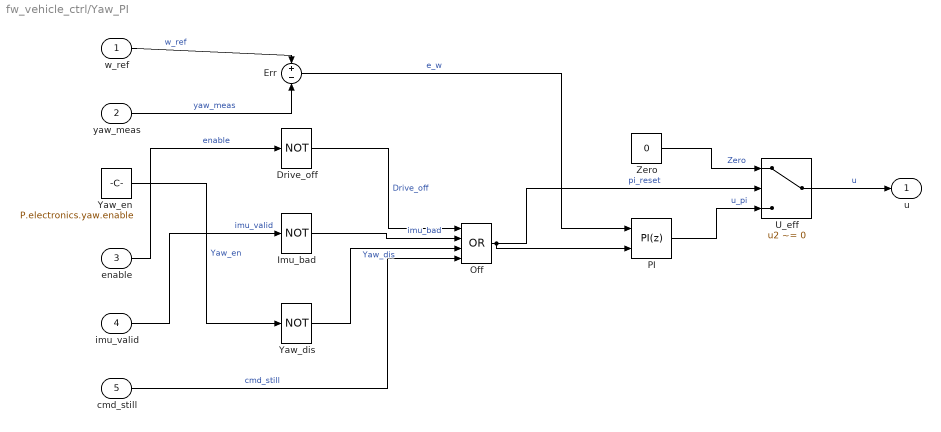
== system fw_vehicle_ctrl/Yaw_PI ==
  w_ref : Inport
  yaw_meas : Inport  Port=2
  enable : Inport  Port=3
  imu_valid : Inport  Port=4
  cmd_still : Inport  Port=5
  Drive_off : Logic  Operator=NOT  Inputs=1  AllPortsSameDT=off  OutDataTypeStr=boolean
  Err : Sum  Inputs=+-
  Imu_bad : Logic  Operator=NOT  Inputs=1  AllPortsSameDT=off  OutDataTypeStr=boolean
  Off : Logic  Operator=OR  Inputs=4  AllPortsSameDT=off  OutDataTypeStr=boolean
  PI : slpidlib/PID Controller  Controller=PI  Form=Parallel  TimeDomain=Discrete-time  UseExternalTs=off  SampleTime=Ts.ctrl  IntegratorMethod=Forward Euler  FilterMethod=Forward Euler  ControllerParametersSource=internal  P=P.electronics.yaw.Kp  I=P.electronics.yaw.Ki  UseKiTs=off  D=0  UseExternalDerivativeSource=off  N=100  UseFilter=on  TunerSelectOption=Transfer Function Based (PID Tuner App)  InitialConditionSource=internal  InitialConditionForIntegrator=0  InitialConditionForFilter=0  DifferentiatorICPrevScaledInput=0  ExternalReset=level  TrackingMode=off  Kt=1  LimitOutput=on  SatLimitsSource=internal  UpperSaturationLimit=P.electronics.yaw.u_max  LowerSaturationLimit=-P.electronics.yaw.u_max  LinearizeAsGain=off  AntiWindupMode=clamping  Kb=1  LimitIntegrator=off  UpperIntegratorSaturationLimit=inf  LowerIntegratorSaturationLimit=-inf  POutMin=[]  POutMax=[]  IOutMin=[]  IOutMax=[]  DOutMin=[]  DOutMax=[]  NOutMin=[]  NOutMax=[]  SumOutMin=[]  SumOutMax=[]  SaturationOutMin=[]  SaturationOutMax=[]  PParamMin=[]  PParamMax=[]  IParamMin=[]  IParamMax=[]  DParamMin=[]  DParamMax=[]  NParamMin=[]  NParamMax=[]  KbParamMin=[]  KbParamMax=[]  KtParamMin=[]  KtParamMax=[]  KbOutMin=[]  KbOutMax=[]  KtOutMin=[]  KtOutMax=[]  IntegratorOutMin=[]  IntegratorOutMax=[]  FilterOutMin=[]  FilterOutMax=[]  SumI1OutMin=[]  SumI1OutMax=[]  SumI2OutMin=[]  SumI2OutMax=[]  SumI3OutMin=[]  SumI3OutMax=[]  SumI4OutMin=[]  SumI4OutMax=[]  SumDOutMin=[]  SumDOutMax=[]  DifferentiatorOutMin=[]  DifferentiatorOutMax=[]  FilterDiffOutCoefMin=[]  FilterDiffOutCoefMax=[]  ReciprocalOutMin=[]  ReciprocalOutMax=[]  SumDenOutMin=[]  SumDenOutMax=[]  SumNumOutMin=[]  SumNumOutMax=[]  DivideOutMin=[]  DivideOutMax=[]  UdiffTsProdOutMin=[]  UdiffTsProdOutMax=[]  NTsProdOutMin=[]  NTsProdOutMax=[]  UintegralTsProdOutMin=[]  UintegralTsProdOutMax=[]  UngainTsProdOutMin=[]  UngainTsProdOutMax=[]  ClampingZeroOutDataTypeStr=Inherit: Inherit via back propagation  ClampingZeroOutMin=[]  ClampingZeroOutMax=[]  FilterDenConstantOutDataTypeStr=Inherit: Inherit via back propagation  FilterDenConstantOutMin=[]  FilterDenConstantOutMax=[]  PCopyOutDataTypeStr=Inherit: Inherit via back propagation  PCopyOutMin=[]  PCopyOutMax=[]  NCopyOutDataTypeStr=Inherit: Inherit via back propagation  NCopyOutMin=[]  NCopyOutMax=[]  IntegratorContinuousStateAttributes=''  IntegratorStateMustResolveToSignalObject=off  IntegratorRTWStateStorageClass=Auto  FilterContinuousStateAttributes=''  FilterStateMustResolveToSignalObject=off  FilterRTWStateStorageClass=Auto  ParallelPVariant=InternalParameters  IdealPVariant=Disabled  IVariant=InternalParameters  DVariant=Disabled  IntegratorVariant=Discrete  SatVariant=Enabled  AWVariant=DiscClampingParallel  PCopyVariant=Disabled  TRVariant=Disabled  FdbkBlocksVariant=Forward  IdealPFdbkVariant=Disabled  SatFdbkVariant=Disabled  DerivativeFilterVariant=Disabled  NVariant=Disabled  NCopyVariant=Disabled_SignalSpec  FilterICVariant=Disabled  IntegratorICVariant=InternalICs  ExternalResetVariant=ExternalReset  TRSumVariant=Passthrough  SumFdbkVariant=Disabled  SumVariant=Sum_PI  TsampFilterVariant=InternalTs  TsampNgainVariant=Passthrough  TsampIntegralVariant=Disabled_SignalSpec  ExternalSaturationOutDataTypeStr=Inherit: Same as second input  DerivativeSourceVariant=Disabled  PreIntVariant=InternalPreInt
      settings: LibrarySourceBlock=simulink/Discrete/Discrete PID Controller
  U_eff : Switch  Criteria=u2 ~= 0  SaturateOnIntegerOverflow=off  InputSameDT=off
  Yaw_dis : Logic  Operator=NOT  Inputs=1  AllPortsSameDT=off  OutDataTypeStr=boolean
  Yaw_en : Constant  Value=P.electronics.yaw.enable  OutDataTypeStr=boolean  SampleTime=Ts.ctrl
  Zero : Constant  Value=0  OutDataTypeStr=single  SampleTime=Ts.ctrl
  u : Outport
  wires:
  w_ref/1 -> Err/1  "w_ref"
  yaw_meas/1 -> Err/2  "yaw_meas"
  Yaw_en/1 -> Yaw_dis/1  "Yaw_en"
  enable/1 -> Drive_off/1  "enable"
  imu_valid/1 -> Imu_bad/1  "imu_valid"
  cmd_still/1 -> Off/4  "cmd_still"
  Err/1 -> PI/1  "e_w"
  Drive_off/1 -> Off/1  "Drive_off"
  Imu_bad/1 -> Off/2  "imu_bad"
  Yaw_dis/1 -> Off/3  "Yaw_dis"
  Off/1 -> U_eff/2, PI/2  "pi_reset"
  Zero/1 -> U_eff/1  "Zero"
  PI/1 -> U_eff/3  "u_pi"
  U_eff/1 -> u/1  "u"

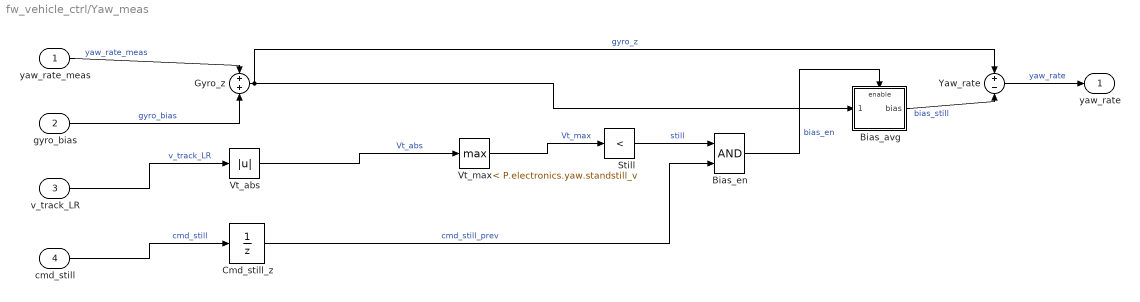
== system fw_vehicle_ctrl/Yaw_meas ==
  yaw_rate_meas : Inport
  gyro_bias : Inport  Port=2
  v_track_LR : Inport  Port=3
  cmd_still : Inport  Port=4
  Bias_avg : Subsystem
  Bias_en : Logic  AllPortsSameDT=off  OutDataTypeStr=boolean
  Cmd_still_z : UnitDelay  SampleTime=-1
  Gyro_z : Sum
  Still : simulink/Logic and Bit Operations/Compare To Constant  relop=<  const=P.electronics.yaw.standstill_v  OutDataTypeStr=boolean
  Vt_abs : Abs  SaturateOnIntegerOverflow=off
  Vt_max : MinMax  Function=max
  Yaw_rate : Sum  Inputs=+-
  yaw_rate : Outport
  wires:
  yaw_rate_meas/1 -> Gyro_z/1  "yaw_rate_meas"
  gyro_bias/1 -> Gyro_z/2  "gyro_bias"
  v_track_LR/1 -> Vt_abs/1  "v_track_LR"
  cmd_still/1 -> Cmd_still_z/1  "cmd_still"
  Gyro_z/1 -> Bias_avg/1(gyro_z), Yaw_rate/1  "gyro_z"
  Vt_abs/1 -> Vt_max/1  "Vt_abs"
  Cmd_still_z/1 -> Bias_en/2  "cmd_still_prev"
  Vt_max/1 -> Still/1  "Vt_max"
  Still/1 -> Bias_en/1  "still"
  Bias_en/1 -> Bias_avg/Enable  "bias_en"
  Bias_avg/1(bias) -> Yaw_rate/2  "bias_still"
  Yaw_rate/1 -> yaw_rate/1  "yaw_rate"

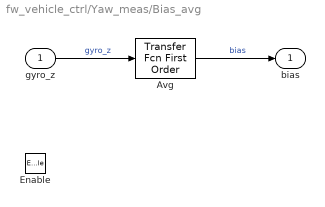
== system fw_vehicle_ctrl/Yaw_meas/Bias_avg ==
  gyro_z : Inport
  Enable : EnablePort
  Avg : simulink/Discrete/Transfer Fcn First Order  PoleZ=exp(-Ts.ctrl/P.electronics.yaw.tau_bias)  ICPrevOutput=0  DoSatur=off
  bias : Outport  InitialOutput=0
  wires:
  gyro_z/1 -> Avg/1  "gyro_z"
  Avg/1 -> bias/1  "bias"
